simulink model "AvonGasTurbineFAult"  (R2016b)
settings: Solver=ode45  StartTime=0.0  StopTime=3000  FixedStep=1  RelTol=1e-3  EnableMultiTasking=on
InitFcn:
  | warning off
undefined symbols (not defined in the file or in its folder): flagFalut, thresholdbound, xflt
libraries: neural x74, fuzblock x6, simulink x5
(part 4 of 4)

== system AvonGasTurbineFAult/exhst temp turbine gg/Layer 1/Delays 1 ==
  "p{1}" : Inport  PortDimensions=4
      mask Display: e = 0.06;c1 = [120 230 180]/255;c2 = ([120 230 180]+0)/(256+128);c3 = ([120 230 180]+128)/(256+128);patch([0 1 1 0],[0 0 1 1],c1);patch([0 1 1 1-e 1-e 0+e],[0 0 1 1-e 0+e 0+e],c2);patch([0 0 1 1-e 0+e 0+e],[0 1 1 1-e 1-e 0+e],c3);plot([0 1 1 0 0],[0 0 1 1 0]);
  mux : Mux  Inputs=1
      mask Display: e = 0.06;c1 = [120 150 230]/255;c2 = ([120 150 230]+0)/383;c3 = ([120 150 230]+128)/383;patch([0 1 1 0],[0 0 1 1],c1);patch([0 1 1 1-e 1-e 0+e],[0 0 1 1-e 0+e 0+e],c2);patch([0 0 1 1-e 0+e 0+e],[0 1 1 1-e 1-e 0+e],c3);plot([0 1 1 0 0],[0 0 1 1 0]);disp('Mux')
  "pd{1,1}" : Outport
      mask Display: e = 0.06;c1 = [120 230 180]/255;c2 = ([120 230 180]+0)/(256+128);c3 = ([120 230 180]+128)/(256+128);patch([0 1 1 0],[0 0 1 1],c1);patch([0 1 1 1-e 1-e 0+e],[0 0 1 1-e 0+e 0+e],c2);patch([0 0 1 1-e 0+e 0+e],[0 1 1 1-e 1-e 0+e],c3);plot([0 1 1 0 0],[0 0 1 1 0]);
  wires:
  "p{1}"/1 -> mux/1
  mux/1 -> "pd{1,1}"/1

== system AvonGasTurbineFAult/exhst temp turbine gg/Layer 1/IW{1,1} ==
  "pd{1,1}" : Inport  PortDimensions=4
      mask Display: e = 0.06;c1 = [120 230 180]/255;c2 = ([120 230 180]+0)/(256+128);c3 = ([120 230 180]+128)/(256+128);patch([0 1 1 0],[0 0 1 1],c1);patch([0 1 1 1-e 1-e 0+e],[0 0 1 1-e 0+e 0+e],c2);patch([0 0 1 1-e 0+e 0+e],[0 1 1 1-e 1-e 0+e],c3);plot([0 1 1 0 0],[0 0 1 1 0]);
  "IW{1,1}(1,:)'" : Constant  Value=[1.2552037635962412;-4.337325079321138;1.2389220325518131;-4.2200588671254069]
      mask Display: e = 0.06;c1 = [120 150 230]/255;c2 = ([120 150 230]+0)/383;c3 = ([120 150 230]+128)/383;patch([0 1 1 0],[0 0 1 1],c1);patch([0 1 1 1-e 1-e 0+e],[0 0 1 1-e 0+e 0+e],c2);patch([0 0 1 1-e 0+e 0+e],[0 1 1 1-e 1-e 0+e],c3);plot([0 1 1 0 0],[0 0 1 1 0]);disp('Weights');
  "IW{1,1}(10,:)'" : Constant  Value=[-3.1457123375316232;-4.0755259466054214;-4.2688288652524173;2.4085329186377415]
      mask Display: e = 0.06;c1 = [120 150 230]/255;c2 = ([120 150 230]+0)/383;c3 = ([120 150 230]+128)/383;patch([0 1 1 0],[0 0 1 1],c1);patch([0 1 1 1-e 1-e 0+e],[0 0 1 1-e 0+e 0+e],c2);patch([0 0 1 1-e 0+e 0+e],[0 1 1 1-e 1-e 0+e],c3);plot([0 1 1 0 0],[0 0 1 1 0]);disp('Weights');
  "IW{1,1}(2,:)'" : Constant  Value=[-0.98779753964890271;-3.1754226877513396;-0.021263476544473775;-4.053488033341103]
      mask Display: e = 0.06;c1 = [120 150 230]/255;c2 = ([120 150 230]+0)/383;c3 = ([120 150 230]+128)/383;patch([0 1 1 0],[0 0 1 1],c1);patch([0 1 1 1-e 1-e 0+e],[0 0 1 1-e 0+e 0+e],c2);patch([0 0 1 1-e 0+e 0+e],[0 1 1 1-e 1-e 0+e],c3);plot([0 1 1 0 0],[0 0 1 1 0]);disp('Weights');
  "IW{1,1}(3,:)'" : Constant  Value=[-0.84171208831296584;-5.1014516495135886;0.86126770483744952;-3.6853675578458525]
      mask Display: e = 0.06;c1 = [120 150 230]/255;c2 = ([120 150 230]+0)/383;c3 = ([120 150 230]+128)/383;patch([0 1 1 0],[0 0 1 1],c1);patch([0 1 1 1-e 1-e 0+e],[0 0 1 1-e 0+e 0+e],c2);patch([0 0 1 1-e 0+e 0+e],[0 1 1 1-e 1-e 0+e],c3);plot([0 1 1 0 0],[0 0 1 1 0]);disp('Weights');
  "IW{1,1}(4,:)'" : Constant  Value=[-5.7526931684897935;-3.8911556528588473;5.334493587141611;1.159530383559823]
      mask Display: e = 0.06;c1 = [120 150 230]/255;c2 = ([120 150 230]+0)/383;c3 = ([120 150 230]+128)/383;patch([0 1 1 0],[0 0 1 1],c1);patch([0 1 1 1-e 1-e 0+e],[0 0 1 1-e 0+e 0+e],c2);patch([0 0 1 1-e 0+e 0+e],[0 1 1 1-e 1-e 0+e],c3);plot([0 1 1 0 0],[0 0 1 1 0]);disp('Weights');
  "IW{1,1}(5,:)'" : Constant  Value=[-1.1644428153610367;2.7048555424010416;-1.7718624058073009;3.7980502485468253]
      mask Display: e = 0.06;c1 = [120 150 230]/255;c2 = ([120 150 230]+0)/383;c3 = ([120 150 230]+128)/383;patch([0 1 1 0],[0 0 1 1],c1);patch([0 1 1 1-e 1-e 0+e],[0 0 1 1-e 0+e 0+e],c2);patch([0 0 1 1-e 0+e 0+e],[0 1 1 1-e 1-e 0+e],c3);plot([0 1 1 0 0],[0 0 1 1 0]);disp('Weights');
  "IW{1,1}(6,:)'" : Constant  Value=[3.2040588304997528;3.8141920263274569;-2.2573635913309169;-9.0812006881940004]
      mask Display: e = 0.06;c1 = [120 150 230]/255;c2 = ([120 150 230]+0)/383;c3 = ([120 150 230]+128)/383;patch([0 1 1 0],[0 0 1 1],c1);patch([0 1 1 1-e 1-e 0+e],[0 0 1 1-e 0+e 0+e],c2);patch([0 0 1 1-e 0+e 0+e],[0 1 1 1-e 1-e 0+e],c3);plot([0 1 1 0 0],[0 0 1 1 0]);disp('Weights');
  "IW{1,1}(7,:)'" : Constant  Value=[-2.7707602705170586;-4.299023534916671;2.9888291828544533;-2.80047451851445]
      mask Display: e = 0.06;c1 = [120 150 230]/255;c2 = ([120 150 230]+0)/383;c3 = ([120 150 230]+128)/383;patch([0 1 1 0],[0 0 1 1],c1);patch([0 1 1 1-e 1-e 0+e],[0 0 1 1-e 0+e 0+e],c2);patch([0 0 1 1-e 0+e 0+e],[0 1 1 1-e 1-e 0+e],c3);plot([0 1 1 0 0],[0 0 1 1 0]);disp('Weights');
  "IW{1,1}(8,:)'" : Constant  Value=[-4.1427143513796452;-4.1811117496581094;2.3378729862330609;0.38144673456814615]
      mask Display: e = 0.06;c1 = [120 150 230]/255;c2 = ([120 150 230]+0)/383;c3 = ([120 150 230]+128)/383;patch([0 1 1 0],[0 0 1 1],c1);patch([0 1 1 1-e 1-e 0+e],[0 0 1 1-e 0+e 0+e],c2);patch([0 0 1 1-e 0+e 0+e],[0 1 1 1-e 1-e 0+e],c3);plot([0 1 1 0 0],[0 0 1 1 0]);disp('Weights');
  "IW{1,1}(9,:)'" : Constant  Value=[1.0609888762345936;-1.1581188357386991;-0.00094914308849244206;-2.0341733864713478]
      mask Display: e = 0.06;c1 = [120 150 230]/255;c2 = ([120 150 230]+0)/383;c3 = ([120 150 230]+128)/383;patch([0 1 1 0],[0 0 1 1],c1);patch([0 1 1 1-e 1-e 0+e],[0 0 1 1-e 0+e 0+e],c2);patch([0 0 1 1-e 0+e 0+e],[0 1 1 1-e 1-e 0+e],c3);plot([0 1 1 0 0],[0 0 1 1 0]);disp('Weights');
  Mux : Mux  Inputs=10
      mask Display: e = 0.06;c1 = [120 150 230]/255;c2 = ([120 150 230]+0)/383;c3 = ([120 150 230]+128)/383;patch([0 1 1 0],[0 0 1 1],c1);patch([0 1 1 1-e 1-e 0+e],[0 0 1 1-e 0+e 0+e],c2);patch([0 0 1 1-e 0+e 0+e],[0 1 1 1-e 1-e 0+e],c3);plot([0 1 1 0 0],[0 0 1 1 0]);disp('Mux');
  dotprod{1..10} (10 alike) : neural/Weight Functions/dotprod
  "iz{1,1}" : Outport
      mask Display: e = 0.06;c1 = [120 230 180]/255;c2 = ([120 230 180]+0)/(256+128);c3 = ([120 230 180]+128)/(256+128);patch([0 1 1 0],[0 0 1 1],c1);patch([0 1 1 1-e 1-e 0+e],[0 0 1 1-e 0+e 0+e],c2);patch([0 0 1 1-e 0+e 0+e],[0 1 1 1-e 1-e 0+e],c3);plot([0 1 1 0 0],[0 0 1 1 0]);
  wires:
  "IW{1,1}(1,:)'"/1 -> dotprod1/1
  "pd{1,1}"/1 -> dotprod1/2, dotprod2/2, dotprod3/2, dotprod4/2, dotprod5/2, dotprod6/2, dotprod7/2, dotprod8/2, dotprod9/2, dotprod10/2
  dotprod1/1 -> Mux/1
  "IW{1,1}(2,:)'"/1 -> dotprod2/1
  dotprod2/1 -> Mux/2
  "IW{1,1}(3,:)'"/1 -> dotprod3/1
  dotprod3/1 -> Mux/3
  "IW{1,1}(4,:)'"/1 -> dotprod4/1
  dotprod4/1 -> Mux/4
  "IW{1,1}(5,:)'"/1 -> dotprod5/1
  dotprod5/1 -> Mux/5
  "IW{1,1}(6,:)'"/1 -> dotprod6/1
  dotprod6/1 -> Mux/6
  "IW{1,1}(7,:)'"/1 -> dotprod7/1
  dotprod7/1 -> Mux/7
  "IW{1,1}(8,:)'"/1 -> dotprod8/1
  dotprod8/1 -> Mux/8
  "IW{1,1}(9,:)'"/1 -> dotprod9/1
  dotprod9/1 -> Mux/9
  "IW{1,1}(10,:)'"/1 -> dotprod10/1
  dotprod10/1 -> Mux/10
  Mux/1 -> "iz{1,1}"/1

== system AvonGasTurbineFAult/exhst temp turbine gg/Layer 2/Delays 1 ==
  "p{2}" : Inport  PortDimensions=10
      mask Display: e = 0.06;c1 = [120 230 180]/255;c2 = ([120 230 180]+0)/(256+128);c3 = ([120 230 180]+128)/(256+128);patch([0 1 1 0],[0 0 1 1],c1);patch([0 1 1 1-e 1-e 0+e],[0 0 1 1-e 0+e 0+e],c2);patch([0 0 1 1-e 0+e 0+e],[0 1 1 1-e 1-e 0+e],c3);plot([0 1 1 0 0],[0 0 1 1 0]);
  mux : Mux  Inputs=1
      mask Display: e = 0.06;c1 = [120 150 230]/255;c2 = ([120 150 230]+0)/383;c3 = ([120 150 230]+128)/383;patch([0 1 1 0],[0 0 1 1],c1);patch([0 1 1 1-e 1-e 0+e],[0 0 1 1-e 0+e 0+e],c2);patch([0 0 1 1-e 0+e 0+e],[0 1 1 1-e 1-e 0+e],c3);plot([0 1 1 0 0],[0 0 1 1 0]);disp('Mux')
  "pd{2,1}" : Outport
      mask Display: e = 0.06;c1 = [120 230 180]/255;c2 = ([120 230 180]+0)/(256+128);c3 = ([120 230 180]+128)/(256+128);patch([0 1 1 0],[0 0 1 1],c1);patch([0 1 1 1-e 1-e 0+e],[0 0 1 1-e 0+e 0+e],c2);patch([0 0 1 1-e 0+e 0+e],[0 1 1 1-e 1-e 0+e],c3);plot([0 1 1 0 0],[0 0 1 1 0]);
  wires:
  "p{2}"/1 -> mux/1
  mux/1 -> "pd{2,1}"/1

== system AvonGasTurbineFAult/exhst temp turbine gg/Layer 2/LW{2,1} ==
  "ad{2,1}" : Inport  PortDimensions=10
      mask Display: e = 0.06;c1 = [120 230 180]/255;c2 = ([120 230 180]+0)/(256+128);c3 = ([120 230 180]+128)/(256+128);patch([0 1 1 0],[0 0 1 1],c1);patch([0 1 1 1-e 1-e 0+e],[0 0 1 1-e 0+e 0+e],c2);patch([0 0 1 1-e 0+e 0+e],[0 1 1 1-e 1-e 0+e],c3);plot([0 1 1 0 0],[0 0 1 1 0]);
  "IW{2,1}(1,:)'" : Constant  Value=[-2.9587960363033265;-4.5827183272957992;-1.4071976182127108;-3.5579824720080686;1.6629956316830536;8.1880706977978033;2.0736267663949182;1.7665060388881453;-2.2799434103503255;-1.108827893431944]
      mask Display: e = 0.06;c1 = [120 150 230]/255;c2 = ([120 150 230]+0)/383;c3 = ([120 150 230]+128)/383;patch([0 1 1 0],[0 0 1 1],c1);patch([0 1 1 1-e 1-e 0+e],[0 0 1 1-e 0+e 0+e],c2);patch([0 0 1 1-e 0+e 0+e],[0 1 1 1-e 1-e 0+e],c3);plot([0 1 1 0 0],[0 0 1 1 0]);disp('weights');
  "IW{2,1}(2,:)'" : Constant  Value=[-6.8388841122057622;6.4531494018104407;-3.5214515018689663;-3.3760802093272368;-4.4501564822453172;-0.025681970245457913;1.6022319320354079;1.0818290916201743;-2.4128514288225618;-4.9486400108650441]
      mask Display: e = 0.06;c1 = [120 150 230]/255;c2 = ([120 150 230]+0)/383;c3 = ([120 150 230]+128)/383;patch([0 1 1 0],[0 0 1 1],c1);patch([0 1 1 1-e 1-e 0+e],[0 0 1 1-e 0+e 0+e],c2);patch([0 0 1 1-e 0+e 0+e],[0 1 1 1-e 1-e 0+e],c3);plot([0 1 1 0 0],[0 0 1 1 0]);disp('weights');
  "IW{2,1}(3,:)'" : Constant  Value=[5.7540044087337288;0.081566457575555001;-6.5054657225367487;-3.1032514337775923;-3.2928093842956447;-0.43818294627670434;-1.6471145238602436;-2.5029353496240088;-1.3040301757611934;4.1162717486777449]
      mask Display: e = 0.06;c1 = [120 150 230]/255;c2 = ([120 150 230]+0)/383;c3 = ([120 150 230]+128)/383;patch([0 1 1 0],[0 0 1 1],c1);patch([0 1 1 1-e 1-e 0+e],[0 0 1 1-e 0+e 0+e],c2);patch([0 0 1 1-e 0+e 0+e],[0 1 1 1-e 1-e 0+e],c3);plot([0 1 1 0 0],[0 0 1 1 0]);disp('weights');
  "IW{2,1}(4,:)'" : Constant  Value=[2.6954726719449047;-2.5840768266660126;6.8746886396970392;2.6172819923161983;0.43049674313685138;-2.0255466890574425;-5.1491099782742467;-5.4071295117314317;1.0306285727007911;4.0410125019298926]
      mask Display: e = 0.06;c1 = [120 150 230]/255;c2 = ([120 150 230]+0)/383;c3 = ([120 150 230]+128)/383;patch([0 1 1 0],[0 0 1 1],c1);patch([0 1 1 1-e 1-e 0+e],[0 0 1 1-e 0+e 0+e],c2);patch([0 0 1 1-e 0+e 0+e],[0 1 1 1-e 1-e 0+e],c3);plot([0 1 1 0 0],[0 0 1 1 0]);disp('weights');
  "IW{2,1}(5,:)'" : Constant  Value=[0.45888374876803506;0.97428796419023644;1.8655228351417508;6.2637784935719392;3.6852846398042751;-4.9419557459874808;3.4410510588521839;4.0781788868249214;3.468050861851852;-1.3742350111265347]
      mask Display: e = 0.06;c1 = [120 150 230]/255;c2 = ([120 150 230]+0)/383;c3 = ([120 150 230]+128)/383;patch([0 1 1 0],[0 0 1 1],c1);patch([0 1 1 1-e 1-e 0+e],[0 0 1 1-e 0+e 0+e],c2);patch([0 0 1 1-e 0+e 0+e],[0 1 1 1-e 1-e 0+e],c3);plot([0 1 1 0 0],[0 0 1 1 0]);disp('weights');
  Mux : Mux  Inputs=5
      mask Display: e = 0.06;c1 = [120 150 230]/255;c2 = ([120 150 230]+0)/383;c3 = ([120 150 230]+128)/383;patch([0 1 1 0],[0 0 1 1],c1);patch([0 1 1 1-e 1-e 0+e],[0 0 1 1-e 0+e 0+e],c2);patch([0 0 1 1-e 0+e 0+e],[0 1 1 1-e 1-e 0+e],c3);plot([0 1 1 0 0],[0 0 1 1 0]);disp('Mux');
  dotprod{1..5} (5 alike) : neural/Weight Functions/dotprod
  "lz{2,1}" : Outport
      mask Display: e = 0.06;c1 = [120 230 180]/255;c2 = ([120 230 180]+0)/(256+128);c3 = ([120 230 180]+128)/(256+128);patch([0 1 1 0],[0 0 1 1],c1);patch([0 1 1 1-e 1-e 0+e],[0 0 1 1-e 0+e 0+e],c2);patch([0 0 1 1-e 0+e 0+e],[0 1 1 1-e 1-e 0+e],c3);plot([0 1 1 0 0],[0 0 1 1 0]);
  wires:
  "IW{2,1}(1,:)'"/1 -> dotprod1/1
  "ad{2,1}"/1 -> dotprod1/2, dotprod2/2, dotprod3/2, dotprod4/2, dotprod5/2
  dotprod1/1 -> Mux/1
  "IW{2,1}(2,:)'"/1 -> dotprod2/1
  dotprod2/1 -> Mux/2
  "IW{2,1}(3,:)'"/1 -> dotprod3/1
  dotprod3/1 -> Mux/3
  "IW{2,1}(4,:)'"/1 -> dotprod4/1
  dotprod4/1 -> Mux/4
  "IW{2,1}(5,:)'"/1 -> dotprod5/1
  dotprod5/1 -> Mux/5
  Mux/1 -> "lz{2,1}"/1

== system AvonGasTurbineFAult/Subsystem/Combustor/combustion chamber 1/ Cp dry air  ==
  Tinlet : Inport
  Cp : Fcn  Expr=(3.355+5.75*1e-4*u(1)-1600*u(1)^(-2))*0.28714  SampleTime=1
  Cp(T) : Outport
  wires:
  Tinlet/1 -> Cp/1
  Cp/1 -> Cp(T)/1

== system AvonGasTurbineFAult/Subsystem/Combustor/combustion chamber 1/Cp Hot Gas  ==
  Tinlet : Inport
  Cp : Fcn  Expr=(3.355+5.75*1e-4*u(1)-1600*u(1)^(-2))*0.28714  SampleTime=1
  Cp(T) : Outport
  wires:
  Tinlet/1 -> Cp/1  "Kelvin"
  Cp/1 -> Cp(T)/1

== system AvonGasTurbineFAult/Subsystem/Combustor/combustion chamber 1/Cp fuel ==
  Tinlet : Inport
  Cp : Fcn  Expr=(1.702+9.081*1e-3*u(1)-2.164*1e-6*u(1)^2)*0.5183  SampleTime=1
  oC-----> K : Fcn  Expr=(u(1)+273.15)  SampleTime=1
  Cp(T) : Outport
  wires:
  oC-----> K/1 -> Cp/1
  Cp/1 -> Cp(T)/1
  Tinlet/1 -> oC-----> K/1

== system AvonGasTurbineFAult/Subsystem/FG MCV model/CV model chamber 2/Cp FG ==
  Tinlet : Inport
  Cp : Fcn  Expr=(1.702+9.081*1e-3*u(1)-2.164*1e-6*u(1)^2)*0.5183  SampleTime=1
  oC-----> K : Fcn  Expr=(u(1)+273.15)  SampleTime=1
  Cp(T) : Outport
  wires:
  oC-----> K/1 -> Cp/1
  Cp/1 -> Cp(T)/1
  Tinlet/1 -> oC-----> K/1

== system AvonGasTurbineFAult/Subsystem/FG MCV model/CV model chamber 2/density FG ==
  FG_prss : Inport
  FG_temp : Inport  Port=2
  1+0.257*Pr-0.533*Pr/Tr : Fcn  Expr=1+0.257*u(1)-0.533*u(1)/u(2)
  Constant3 : Constant  Value=273.15
  Mux : Mux  Inputs=2
  Sum2 : Sum  Inputs=|++
  Tcr : Constant  Value=191
  Tnormal : Constant  Value=273.15+15
  Tnormal/T : Product  Inputs=*/  RndMeth=Zero
  Zn : Constant  Value=0.9974
  density @ n.c.1 : Gain  Gain=0.78862
  density @ n.c.2 : Gain  Gain=1/14.89
  p/pcr : Product  Inputs=*/  RndMeth=Zero
  p/pnormal1 : Product  Inputs=/*  RndMeth=Zero
  p1 : Product  Inputs=3  RndMeth=Zero
  pcr : Constant  Value=4640
  pnormal2 : Constant  Value=101.3
  t/Tc : Product  Inputs=*/  RndMeth=Zero
  z correction : Product  Inputs=/*  RndMeth=Zero
  density : Outport
  wires:
  Tnormal/1 -> Tnormal/T/1
  Constant3/1 -> Sum2/2
  Sum2/1 -> Tnormal/T/2, t/Tc/1
  pcr/1 -> p/pcr/2
  Tcr/1 -> t/Tc/2
  Zn/1 -> z correction/2
  FG_temp/1 -> Sum2/1
  p/pcr/1 -> Mux/1  "pr"
  t/Tc/1 -> Mux/2  "Tr"
  density @ n.c.2/1 -> density/1
  z correction/1 -> p1/3
  Mux/1 -> 1+0.257*Pr-0.533*Pr/Tr/1
  1+0.257*Pr-0.533*Pr/Tr/1 -> z correction/1
  FG_prss/1 -> p/pnormal1/2, p/pcr/1
  pnormal2/1 -> p/pnormal1/1
  p/pnormal1/1 -> p1/2
  p1/1 -> density @ n.c.1/1
  density @ n.c.1/1 -> density @ n.c.2/1
  Tnormal/T/1 -> p1/1

== system AvonGasTurbineFAult/Subsystem/FG MCV model/Subsystem1/Z ==
  T : Inport
  P : Inport  Port=2
  1+0.257*Pr-0.533*Pr/Tr1 : Fcn  Expr=1+0.257*u(1)-0.533*u(1)/u(2)
  Mux5 : Mux  Inputs=2
  Tcr1 : Constant  Value=191
  p/pcr1 : Product  Inputs=*/  RndMeth=Zero
  pcr1 : Constant  Value=4640
  t/Tc1 : Product  Inputs=*/  RndMeth=Zero
  Z : Outport
  wires:
  Mux5/1 -> 1+0.257*Pr-0.533*Pr/Tr1/1
  P/1 -> p/pcr1/1
  T/1 -> t/Tc1/1
  Tcr1/1 -> t/Tc1/2
  1+0.257*Pr-0.533*Pr/Tr1/1 -> Z/1
  t/Tc1/1 -> Mux5/2  "Tr"
  pcr1/1 -> p/pcr1/2
  p/pcr1/1 -> Mux5/1  "pr"

== system AvonGasTurbineFAult/Subsystem/Subsystem1/Turbine section/hot_air ==
  Tinlet : Inport
  Cp(T) : Fcn  Expr=(3.355+5.75*1e-4*u(1)-1600*u(1)^(-2))*0.28714  SampleTime=1
  Cp(P1,T1) : Outport
  wires:
  Tinlet/1 -> Cp(T)/1
  Cp(T)/1 -> Cp(P1,T1)/1

== system AvonGasTurbineFAult/Subsystem/Subsystem2/Turbine section/hot_air ==
  Tinlet : Inport
  Cp(T) : Fcn  Expr=(3.355+5.75*1e-4*u(1)-1600*u(1)^(-2))*0.28714  SampleTime=1
  Cp(P1,T1) : Outport
  wires:
  Cp(T)/1 -> Cp(P1,T1)/1
  Tinlet/1 -> Cp(T)/1

== system AvonGasTurbineFAult/Subsystem/Subsystem2/cooling 1/Cp Temp ==
  Tinlet : Inport
  Cp : Fcn  Expr=(3.355+5.75*1e-4*u(1)-1600*u(1)^(-2))*0.28714  SampleTime=1
  Cp(T) : Outport
  wires:
  Cp/1 -> Cp(T)/1
  Tinlet/1 -> Cp/1  "Kelvin"

== system AvonGasTurbineFAult/Subsystem/Subsystem2/cooling 1/Cp Temp air ==
  Tinlet : Inport
  Cp : Fcn  Expr=(3.355+5.75*1e-4*u(1)-1600*u(1)^(-2))*0.28714  SampleTime=1
  Cp(T) : Outport
  wires:
  Tinlet/1 -> Cp/1  "Kelvin"
  Cp/1 -> Cp(T)/1

== system AvonGasTurbineFAult/Subsystem/Subsystem2/cooling 1/Cp Temp hot gas ==
  Tinlet : Inport
  Cp : Fcn  Expr=(3.355+5.75*1e-4*u(1)-1600*u(1)^(-2))*0.28714  SampleTime=1
  Cp(T) : Outport
  wires:
  Cp/1 -> Cp(T)/1
  Tinlet/1 -> Cp/1  "Kelvin"

== system AvonGasTurbineFAult/Subsystem/Subsystem2/cooling 2/Cp Temp ==
  Tinlet : Inport
  Cp : Fcn  Expr=(3.355+5.75*1e-4*u(1)-1600*u(1)^(-2))*0.28714  SampleTime=1
  Cp(T) : Outport
  wires:
  Tinlet/1 -> Cp/1  "Kelvin"
  Cp/1 -> Cp(T)/1

== system AvonGasTurbineFAult/Subsystem/Subsystem2/cooling 2/Cp Temp air ==
  Tinlet : Inport
  Cp : Fcn  Expr=(3.355+5.75*1e-4*u(1)-1600*u(1)^(-2))*0.28714  SampleTime=1
  Cp(T) : Outport
  wires:
  Cp/1 -> Cp(T)/1
  Tinlet/1 -> Cp/1  "Kelvin"

== system AvonGasTurbineFAult/Subsystem/Subsystem2/cooling 2/Cp Temp hot gas ==
  Tinlet : Inport
  Cp : Fcn  Expr=(3.355+5.75*1e-4*u(1)-1600*u(1)^(-2))*0.28714  SampleTime=1
  Cp(T) : Outport
  wires:
  Tinlet/1 -> Cp/1  "Kelvin"
  Cp/1 -> Cp(T)/1

== system AvonGasTurbineFAult/Subsystem/comp_temp/Cp_com_in/Cp dry air ==
  Tinlet : Inport
  Cp : Fcn  Expr=(3.355+5.75*1e-4*u(1)-1600*u(1)^(-2))*0.28714  SampleTime=1
  Cp(T) : Outport
  wires:
  Cp/1 -> Cp(T)/1
  Tinlet/1 -> Cp/1

== system AvonGasTurbineFAult/Subsystem/comp_temp/Cp_com_in/Cp steam ==
  Tinlet : Inport
  Cp : Fcn  Expr=(3.47+1.45*1e-3*u(1)+1.21*1e4*u(1)^(-2))*0.4615  SampleTime=1
  Cp(T) : Outport
  wires:
  Tinlet/1 -> Cp/1
  Cp/1 -> Cp(T)/1

== system AvonGasTurbineFAult/Subsystem/comp_temp/Cp_com_in/Specific humidity ==
  humidity : Inport
  Press_kPa : Inport  Port=2
  temp : Inport  Port=3
  1/100 : Gain  Gain=0.01
  Ps (saturation pressure) : Fcn  Expr=((u-200.5754)/81.4934)^6.1556  SampleTime=1
  Scope11 : Scope
  "Specific humidity " : Gain  Gain=0.6219
  Sum : Sum  Inputs=-+
  x : Product  RndMeth=Zero
  x1 : Product  Inputs=*/  RndMeth=Zero
  y : Outport
  wires:
  Ps (saturation pressure)/1 -> Scope11/1, x/1
  "Specific humidity "/1 -> y/1
  x1/1 -> "Specific humidity "/1
  Sum/1 -> x1/2
  Press_kPa/1 -> Sum/2
  x/1 -> x1/1, Sum/1  "pv"
  1/100/1 -> x/2
  humidity/1 -> 1/100/1
  temp/1 -> Ps (saturation pressure)/1
